simulink model "skarab_adc4x3g_14_byp"  (R2018a)
settings: Solver=VariableStepAuto  StartTime=0.0  StopTime=10.0  RelTol=1e-3
libraries: xbsIndex_r4 x140
settings Model: Creator=aisaacson  LastModifiedBy=clifford

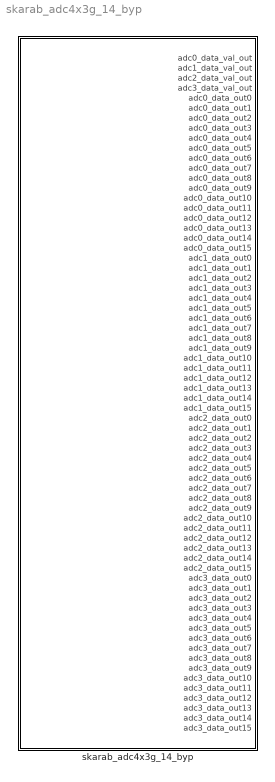
== system skarab_adc4x3g_14_byp ==
  skarab_adc4x3g_14_byp : Subsystem  Tag=xps:skarab_adc4x3g_14_byp  mask(hmc){mez=2, sync_ms=Master}
      mask prompts: mez "Mezzanine slot"; sync_ms "Master/Slave"
      mask help: Interface to ADC cards available on SKARAB boards.
      mask init:
      | skarab_adc4x3g_14_byp_mask(gcb);
      mask TypeOptions mez: 0 | 1 | 2 | 3
      mask TypeOptions sync_ms: Master | Slave
      mask DialogControl Container6 Prompt: Parameters

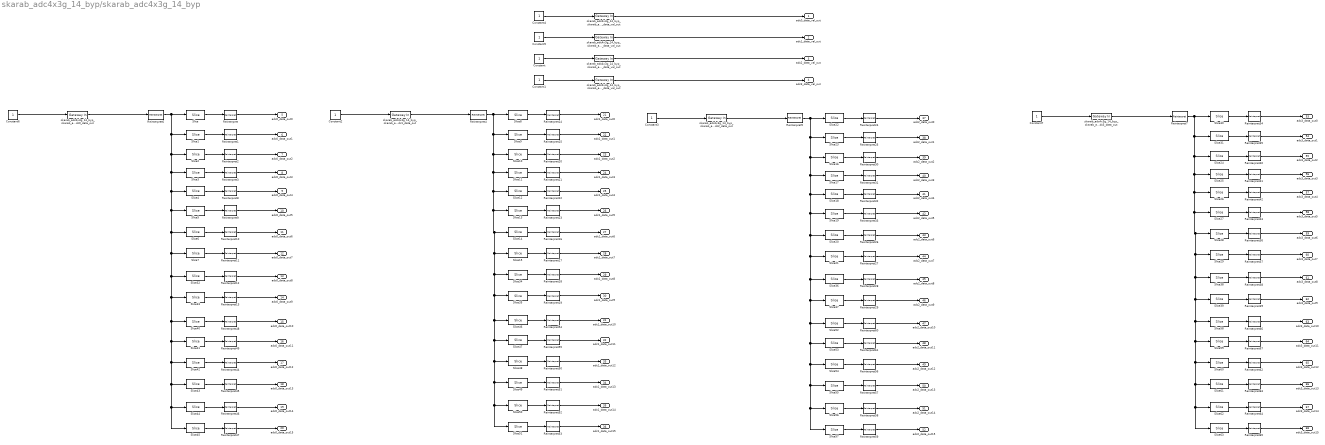
== system skarab_adc4x3g_14_byp/skarab_adc4x3g_14_byp ==
  Constant{,1..7} (8 alike) : Constant
  Reinterpret{,1..3,8..67} (64 alike) : xbsIndex_r4/Reinterpret  force_arith_type=on  arith_type="Signed  (2's comp)"  force_bin_pt=on  bin_pt=11  block_type=reinterpret
  Reinterpret{4..7} (4 alike) : xbsIndex_r4/Reinterpret  force_arith_type=on  arith_type=Unsigned  force_bin_pt=on  bin_pt=0  block_type=reinterpret
  Slice{,8,22,30} (4 alike) : xbsIndex_r4/Slice  nbits=12  boolean_output=off  mode=Lower Bit Location + Width  bit1=0  base1=MSB of Input  bit0=0  base0=LSB of Input  dbl_ovrd=off  block_type=slice
  Slice{1,9,23,31} (4 alike) : xbsIndex_r4/Slice  nbits=12  boolean_output=off  mode=Lower Bit Location + Width  bit1=0  base1=MSB of Input  bit0=12  base0=LSB of Input  dbl_ovrd=off  block_type=slice
  Slice{2,10,16,24} (4 alike) : xbsIndex_r4/Slice  nbits=12  boolean_output=off  mode=Lower Bit Location + Width  bit1=0  base1=MSB of Input  bit0=24  base0=LSB of Input  dbl_ovrd=off  block_type=slice
  Slice{3,11,17,25} (4 alike) : xbsIndex_r4/Slice  nbits=12  boolean_output=off  mode=Lower Bit Location + Width  bit1=0  base1=MSB of Input  bit0=36  base0=LSB of Input  dbl_ovrd=off  block_type=slice
  Slice{4,12,18,26} (4 alike) : xbsIndex_r4/Slice  nbits=12  boolean_output=off  mode=Lower Bit Location + Width  bit1=0  base1=MSB of Input  bit0=48  base0=LSB of Input  dbl_ovrd=off  block_type=slice
  Slice{5,13,19,27} (4 alike) : xbsIndex_r4/Slice  nbits=12  boolean_output=off  mode=Lower Bit Location + Width  bit1=0  base1=MSB of Input  bit0=60  base0=LSB of Input  dbl_ovrd=off  block_type=slice
  Slice{6,14,20,28} (4 alike) : xbsIndex_r4/Slice  nbits=12  boolean_output=off  mode=Lower Bit Location + Width  bit1=0  base1=MSB of Input  bit0=72  base0=LSB of Input  dbl_ovrd=off  block_type=slice
  Slice{7,15,21,29} (4 alike) : xbsIndex_r4/Slice  nbits=12  boolean_output=off  mode=Lower Bit Location + Width  bit1=0  base1=MSB of Input  bit0=84  base0=LSB of Input  dbl_ovrd=off  block_type=slice
  Slice{32,34,36,38} (4 alike) : xbsIndex_r4/Slice  nbits=12  boolean_output=off  mode=Lower Bit Location + Width  bit1=0  base1=MSB of Input  bit0=96  base0=LSB of Input  dbl_ovrd=off  block_type=slice
  Slice{33,35,37,39} (4 alike) : xbsIndex_r4/Slice  nbits=12  boolean_output=off  mode=Lower Bit Location + Width  bit1=0  base1=MSB of Input  bit0=108  base0=LSB of Input  dbl_ovrd=off  block_type=slice
  Slice{40,46,52,58} (4 alike) : xbsIndex_r4/Slice  nbits=12  boolean_output=off  mode=Lower Bit Location + Width  bit1=0  base1=MSB of Input  bit0=120  base0=LSB of Input  dbl_ovrd=off  block_type=slice
  Slice{41,47,53,59} (4 alike) : xbsIndex_r4/Slice  nbits=12  boolean_output=off  mode=Lower Bit Location + Width  bit1=0  base1=MSB of Input  bit0=132  base0=LSB of Input  dbl_ovrd=off  block_type=slice
  Slice{42,48,54,60} (4 alike) : xbsIndex_r4/Slice  nbits=12  boolean_output=off  mode=Lower Bit Location + Width  bit1=0  base1=MSB of Input  bit0=144  base0=LSB of Input  dbl_ovrd=off  block_type=slice
  Slice{43,49,55,61} (4 alike) : xbsIndex_r4/Slice  nbits=12  boolean_output=off  mode=Lower Bit Location + Width  bit1=0  base1=MSB of Input  bit0=156  base0=LSB of Input  dbl_ovrd=off  block_type=slice
  Slice{44,50,56,62} (4 alike) : xbsIndex_r4/Slice  nbits=12  boolean_output=off  mode=Lower Bit Location + Width  bit1=0  base1=MSB of Input  bit0=168  base0=LSB of Input  dbl_ovrd=off  block_type=slice
  Slice{45,51,57,63} (4 alike) : xbsIndex_r4/Slice  nbits=12  boolean_output=off  mode=Lower Bit Location + Width  bit1=0  base1=MSB of Input  bit0=180  base0=LSB of Input  dbl_ovrd=off  block_type=slice
  skarab_adc4x3g_14_byp_skarab_adc4x3g_14_byp_adc0_data_out : xbsIndex_r4/Gateway In  gui_display_data_type=Fixed-point  arith_type=Unsigned  n_bits=192  bin_pt=0  preci_type=Single  exp_width=8  frac_width=24  rows=1  columns=1  quantization=Truncate  overflow=Wrap  period=1  UseAsADC=off  ADCChannel='1'  interface=None  automatic_assignment=on  address_offset=hex2dec('00')  intf_name=''  intf_description=''  default_value=0  timing_constraint=None  locs_specified=off  LOCs={}  io_standard={}  inherit_from_input=off  hdl_port=on  dbl_ovrd=off  block_type=gatewayin
  skarab_adc4x3g_14_byp_skarab_adc4x3g_14_byp_adc0_data_val_out : xbsIndex_r4/Gateway In  gui_display_data_type=Boolean  arith_type=Boolean  n_bits=16  bin_pt=14  preci_type=Single  exp_width=8  frac_width=24  rows=1  columns=1  quantization="Round  (unbiased: +/- Inf)"  overflow=Saturate  period=1  UseAsADC=off  ADCChannel='1'  interface=None  automatic_assignment=on  address_offset=hex2dec('00')  intf_name=''  intf_description=''  default_value=0  timing_constraint=None  locs_specified=off  LOCs={}  io_standard={}  inherit_from_input=off  hdl_port=on  dbl_ovrd=off  block_type=gatewayin
  skarab_adc4x3g_14_byp_skarab_adc4x3g_14_byp_adc1_data_out : xbsIndex_r4/Gateway In  gui_display_data_type=Fixed-point  arith_type=Unsigned  n_bits=192  bin_pt=0  preci_type=Single  exp_width=8  frac_width=24  rows=1  columns=1  quantization=Truncate  overflow=Wrap  period=1  UseAsADC=off  ADCChannel='1'  interface=None  automatic_assignment=on  address_offset=hex2dec('00')  intf_name=''  intf_description=''  default_value=0  timing_constraint=None  locs_specified=off  LOCs={}  io_standard={}  inherit_from_input=off  hdl_port=on  dbl_ovrd=off  block_type=gatewayin
  skarab_adc4x3g_14_byp_skarab_adc4x3g_14_byp_adc1_data_val_out : xbsIndex_r4/Gateway In  gui_display_data_type=Boolean  arith_type=Boolean  n_bits=16  bin_pt=14  preci_type=Single  exp_width=8  frac_width=24  rows=1  columns=1  quantization="Round  (unbiased: +/- Inf)"  overflow=Saturate  period=1  UseAsADC=off  ADCChannel='1'  interface=None  automatic_assignment=on  address_offset=hex2dec('00')  intf_name=''  intf_description=''  default_value=0  timing_constraint=None  locs_specified=off  LOCs={}  io_standard={}  inherit_from_input=off  hdl_port=on  dbl_ovrd=off  block_type=gatewayin
  skarab_adc4x3g_14_byp_skarab_adc4x3g_14_byp_adc2_data_out : xbsIndex_r4/Gateway In  gui_display_data_type=Fixed-point  arith_type=Unsigned  n_bits=192  bin_pt=0  preci_type=Single  exp_width=8  frac_width=24  rows=1  columns=1  quantization=Truncate  overflow=Wrap  period=1  UseAsADC=off  ADCChannel='1'  interface=None  automatic_assignment=on  address_offset=hex2dec('00')  intf_name=''  intf_description=''  default_value=0  timing_constraint=None  locs_specified=off  LOCs={}  io_standard={}  inherit_from_input=off  hdl_port=on  dbl_ovrd=off  block_type=gatewayin
  skarab_adc4x3g_14_byp_skarab_adc4x3g_14_byp_adc2_data_val_out : xbsIndex_r4/Gateway In  gui_display_data_type=Boolean  arith_type=Boolean  n_bits=16  bin_pt=14  preci_type=Single  exp_width=8  frac_width=24  rows=1  columns=1  quantization="Round  (unbiased: +/- Inf)"  overflow=Saturate  period=1  UseAsADC=off  ADCChannel='1'  interface=None  automatic_assignment=on  address_offset=hex2dec('00')  intf_name=''  intf_description=''  default_value=0  timing_constraint=None  locs_specified=off  LOCs={}  io_standard={}  inherit_from_input=off  hdl_port=on  dbl_ovrd=off  block_type=gatewayin
  skarab_adc4x3g_14_byp_skarab_adc4x3g_14_byp_adc3_data_out : xbsIndex_r4/Gateway In  gui_display_data_type=Fixed-point  arith_type=Unsigned  n_bits=192  bin_pt=0  preci_type=Single  exp_width=8  frac_width=24  rows=1  columns=1  quantization=Truncate  overflow=Wrap  period=1  UseAsADC=off  ADCChannel='1'  interface=None  automatic_assignment=on  address_offset=hex2dec('00')  intf_name=''  intf_description=''  default_value=0  timing_constraint=None  locs_specified=off  LOCs={}  io_standard={}  inherit_from_input=off  hdl_port=on  dbl_ovrd=off  block_type=gatewayin
  skarab_adc4x3g_14_byp_skarab_adc4x3g_14_byp_adc3_data_val_out : xbsIndex_r4/Gateway In  gui_display_data_type=Boolean  arith_type=Boolean  n_bits=16  bin_pt=14  preci_type=Single  exp_width=8  frac_width=24  rows=1  columns=1  quantization="Round  (unbiased: +/- Inf)"  overflow=Saturate  period=1  UseAsADC=off  ADCChannel='1'  interface=None  automatic_assignment=on  address_offset=hex2dec('00')  intf_name=''  intf_description=''  default_value=0  timing_constraint=None  locs_specified=off  LOCs={}  io_standard={}  inherit_from_input=off  hdl_port=on  dbl_ovrd=off  block_type=gatewayin
  adc0_data_val_out : Outport
  adc1_data_val_out : Outport  Port=2
  adc2_data_val_out : Outport  Port=3
  adc3_data_val_out : Outport  Port=4
  adc0_data_out0 : Outport  Port=5
  adc0_data_out1 : Outport  Port=6
  adc0_data_out2 : Outport  Port=7
  adc0_data_out3 : Outport  Port=8
  adc0_data_out4 : Outport  Port=9
  adc0_data_out5 : Outport  Port=10
  adc0_data_out6 : Outport  Port=11
  adc0_data_out7 : Outport  Port=12
  adc0_data_out8 : Outport  Port=13
  adc0_data_out9 : Outport  Port=14
  adc0_data_out10 : Outport  Port=15
  adc0_data_out11 : Outport  Port=16
  adc0_data_out12 : Outport  Port=17
  adc0_data_out13 : Outport  Port=18
  adc0_data_out14 : Outport  Port=19
  adc0_data_out15 : Outport  Port=20
  adc1_data_out0 : Outport  Port=21
  adc1_data_out1 : Outport  Port=22
  adc1_data_out2 : Outport  Port=23
  adc1_data_out3 : Outport  Port=24
  adc1_data_out4 : Outport  Port=25
  adc1_data_out5 : Outport  Port=26
  adc1_data_out6 : Outport  Port=27
  adc1_data_out7 : Outport  Port=28
  adc1_data_out8 : Outport  Port=29
  adc1_data_out9 : Outport  Port=30
  adc1_data_out10 : Outport  Port=31
  adc1_data_out11 : Outport  Port=32
  adc1_data_out12 : Outport  Port=33
  adc1_data_out13 : Outport  Port=34
  adc1_data_out14 : Outport  Port=35
  adc1_data_out15 : Outport  Port=36
  adc2_data_out0 : Outport  Port=37
  adc2_data_out1 : Outport  Port=38
  adc2_data_out2 : Outport  Port=39
  adc2_data_out3 : Outport  Port=40
  adc2_data_out4 : Outport  Port=41
  adc2_data_out5 : Outport  Port=42
  adc2_data_out6 : Outport  Port=43
  adc2_data_out7 : Outport  Port=44
  adc2_data_out8 : Outport  Port=45
  adc2_data_out9 : Outport  Port=46
  adc2_data_out10 : Outport  Port=47
  adc2_data_out11 : Outport  Port=48
  adc2_data_out12 : Outport  Port=49
  adc2_data_out13 : Outport  Port=50
  adc2_data_out14 : Outport  Port=51
  adc2_data_out15 : Outport  Port=52
  adc3_data_out0 : Outport  Port=53
  adc3_data_out1 : Outport  Port=54
  adc3_data_out2 : Outport  Port=55
  adc3_data_out3 : Outport  Port=56
  adc3_data_out4 : Outport  Port=57
  adc3_data_out5 : Outport  Port=58
  adc3_data_out6 : Outport  Port=59
  adc3_data_out7 : Outport  Port=60
  adc3_data_out8 : Outport  Port=61
  adc3_data_out9 : Outport  Port=62
  adc3_data_out10 : Outport  Port=63
  adc3_data_out11 : Outport  Port=64
  adc3_data_out12 : Outport  Port=65
  adc3_data_out13 : Outport  Port=66
  adc3_data_out14 : Outport  Port=67
  adc3_data_out15 : Outport  Port=68
  wires:
  Reinterpret7/1 -> Slice30/1, Slice31/1, Slice24/1, Slice25/1, Slice26/1, Slice27/1, Slice28/1, Slice29/1, Slice38/1, Slice63/1, Slice62/1, Slice61/1, Slice60/1, Slice59/1, Slice58/1, Slice39/1
  Reinterpret54/1 -> adc1_data_out10/1
  Slice7/1 -> Reinterpret11/1
  Slice55/1 -> Reinterpret57/1
  Reinterpret39/1 -> adc3_data_out9/1
  Slice62/1 -> Reinterpret64/1
  Slice28/1 -> Reinterpret36/1
  Slice22/1 -> Reinterpret24/1
  Reinterpret57/1 -> adc2_data_out13/1
  Reinterpret62/1 -> adc3_data_out12/1
  Reinterpret46/1 -> adc0_data_out14/1
  Reinterpret23/1 -> adc1_data_out5/1
  Slice57/1 -> Reinterpret59/1
  skarab_adc4x3g_14_byp_skarab_adc4x3g_14_byp_adc3_data_val_out/1 -> adc3_data_val_out/1
  Slice54/1 -> Reinterpret56/1
  Constant1/1 -> skarab_adc4x3g_14_byp_skarab_adc4x3g_14_byp_adc3_data_val_out/1
  Slice6/1 -> Reinterpret10/1
  skarab_adc4x3g_14_byp_skarab_adc4x3g_14_byp_adc1_data_out/1 -> Reinterpret4/1
  Slice50/1 -> Reinterpret52/1
  Constant/1 -> skarab_adc4x3g_14_byp_skarab_adc4x3g_14_byp_adc2_data_val_out/1
  Reinterpret30/1 -> adc2_data_out2/1
  Reinterpret47/1 -> adc0_data_out15/1
  Slice21/1 -> Reinterpret27/1
  Slice37/1 -> Reinterpret29/1
  Reinterpret49/1 -> adc0_data_out11/1
  Reinterpret14/1 -> adc1_data_out0/1
  Slice15/1 -> Reinterpret17/1
  Reinterpret10/1 -> adc0_data_out6/1
  skarab_adc4x3g_14_byp_skarab_adc4x3g_14_byp_adc2_data_val_out/1 -> adc2_data_val_out/1
  Reinterpret51/1 -> adc1_data_out13/1
  Reinterpret21/1 -> adc1_data_out3/1
  Reinterpret66/1 -> adc3_data_out10/1
  Slice34/1 -> Reinterpret18/1
  Reinterpret60/1 -> adc2_data_out10/1
  Reinterpret48/1 -> adc0_data_out10/1
  Slice59/1 -> Reinterpret67/1
  Reinterpret12/1 -> adc0_data_out8/1
  Constant4/1 -> skarab_adc4x3g_14_byp_skarab_adc4x3g_14_byp_adc0_data_val_out/1
  skarab_adc4x3g_14_byp_skarab_adc4x3g_14_byp_adc0_data_val_out/1 -> adc0_data_val_out/1
  Slice58/1 -> Reinterpret66/1
  skarab_adc4x3g_14_byp_skarab_adc4x3g_14_byp_adc0_data_out/1 -> Reinterpret6/1
  skarab_adc4x3g_14_byp_skarab_adc4x3g_14_byp_adc1_data_val_out/1 -> adc1_data_val_out/1
  Reinterpret34/1 -> adc3_data_out0/1
  Slice11/1 -> Reinterpret21/1
  Slice5/1 -> Reinterpret9/1
  Slice35/1 -> Reinterpret19/1
  Slice4/1 -> Reinterpret8/1
  Reinterpret9/1 -> adc0_data_out5/1
  Reinterpret/1 -> adc0_data_out0/1
  Constant2/1 -> skarab_adc4x3g_14_byp_skarab_adc4x3g_14_byp_adc1_data_out/1
  Reinterpret11/1 -> adc0_data_out7/1
  Slice23/1 -> Reinterpret25/1
  Slice10/1 -> Reinterpret20/1
  Slice45/1 -> Reinterpret47/1
  Slice42/1 -> Reinterpret44/1
  Reinterpret36/1 -> adc3_data_out6/1
  Slice60/1 -> Reinterpret62/1
  Reinterpret19/1 -> adc1_data_out9/1
  Slice14/1 -> Reinterpret16/1
  Constant6/1 -> skarab_adc4x3g_14_byp_skarab_adc4x3g_14_byp_adc0_data_out/1
  Reinterpret35/1 -> adc3_data_out1/1
  skarab_adc4x3g_14_byp_skarab_adc4x3g_14_byp_adc2_data_out/1 -> Reinterpret5/1
  Slice43/1 -> Reinterpret45/1
  Slice30/1 -> Reinterpret34/1
  Slice41/1 -> Reinterpret49/1
  Reinterpret1/1 -> adc0_data_out1/1
  Reinterpret56/1 -> adc2_data_out12/1
  Slice46/1 -> Reinterpret54/1
  Reinterpret58/1 -> adc2_data_out14/1
  Reinterpret16/1 -> adc1_data_out6/1
  Slice24/1 -> Reinterpret40/1
  Reinterpret37/1 -> adc3_data_out7/1
  Constant3/1 -> skarab_adc4x3g_14_byp_skarab_adc4x3g_14_byp_adc2_data_out/1
  Reinterpret5/1 -> Slice22/1, Slice23/1, Slice16/1, Slice17/1, Slice18/1, Slice19/1, Slice20/1, Slice21/1, Slice36/1, Slice57/1, Slice56/1, Slice55/1, Slice54/1, Slice53/1, Slice52/1, Slice37/1
  Slice12/1 -> Reinterpret22/1
  Slice32/1 -> Reinterpret12/1
  Slice13/1 -> Reinterpret23/1
  Reinterpret41/1 -> adc3_data_out3/1
  Reinterpret15/1 -> adc1_data_out1/1
  Reinterpret17/1 -> adc1_data_out7/1
  Reinterpret40/1 -> adc3_data_out2/1
  Slice33/1 -> Reinterpret13/1
  Reinterpret45/1 -> adc0_data_out13/1
  Reinterpret28/1 -> adc2_data_out8/1
  Reinterpret42/1 -> adc3_data_out4/1
  Slice38/1 -> Reinterpret38/1
  Reinterpret38/1 -> adc3_data_out8/1
  Reinterpret22/1 -> adc1_data_out4/1
  Reinterpret43/1 -> adc3_data_out5/1
  Reinterpret25/1 -> adc2_data_out1/1
  Slice2/1 -> Reinterpret2/1
  Reinterpret63/1 -> adc3_data_out13/1
  Slice31/1 -> Reinterpret35/1
  Reinterpret6/1 -> Slice/1, Slice1/1, Slice2/1, Slice3/1, Slice4/1, Slice5/1, Slice6/1, Slice7/1, Slice32/1, Slice45/1, Slice44/1, Slice43/1, Slice42/1, Slice41/1, Slice40/1, Slice33/1
  Slice27/1 -> Reinterpret43/1
  Slice52/1 -> Reinterpret60/1
  Slice39/1 -> Reinterpret39/1
  Slice29/1 -> Reinterpret37/1
  Reinterpret20/1 -> adc1_data_out2/1
  Constant5/1 -> skarab_adc4x3g_14_byp_skarab_adc4x3g_14_byp_adc1_data_val_out/1
  Slice16/1 -> Reinterpret30/1
  Slice8/1 -> Reinterpret14/1
  Slice9/1 -> Reinterpret15/1
  Reinterpret53/1 -> adc1_data_out15/1
  Reinterpret29/1 -> adc2_data_out9/1
  Slice25/1 -> Reinterpret41/1
  Slice/1 -> Reinterpret/1
  Slice51/1 -> Reinterpret53/1
  Slice44/1 -> Reinterpret46/1
  Reinterpret3/1 -> adc0_data_out3/1
  Reinterpret67/1 -> adc3_data_out11/1
  Slice47/1 -> Reinterpret55/1
  Reinterpret2/1 -> adc0_data_out2/1
  skarab_adc4x3g_14_byp_skarab_adc4x3g_14_byp_adc3_data_out/1 -> Reinterpret7/1
  Reinterpret18/1 -> adc1_data_out8/1
  Reinterpret27/1 -> adc2_data_out7/1
  Slice20/1 -> Reinterpret26/1
  Slice1/1 -> Reinterpret1/1
  Slice63/1 -> Reinterpret65/1
  Reinterpret26/1 -> adc2_data_out6/1
  Slice18/1 -> Reinterpret32/1
  Reinterpret13/1 -> adc0_data_out9/1
  Slice19/1 -> Reinterpret33/1
  Slice48/1 -> Reinterpret50/1
  Slice26/1 -> Reinterpret42/1
  Reinterpret33/1 -> adc2_data_out5/1
  Slice56/1 -> Reinterpret58/1
  Reinterpret65/1 -> adc3_data_out15/1
  Reinterpret4/1 -> Slice8/1, Slice9/1, Slice10/1, Slice11/1, Slice12/1, Slice13/1, Slice14/1, Slice15/1, Slice51/1, Slice50/1, Slice49/1, Slice48/1, Slice47/1, Slice46/1, Slice35/1, Slice34/1
  Reinterpret44/1 -> adc0_data_out12/1
  Slice40/1 -> Reinterpret48/1
  Slice61/1 -> Reinterpret63/1
  Reinterpret50/1 -> adc1_data_out12/1
  Slice49/1 -> Reinterpret51/1
  Slice17/1 -> Reinterpret31/1
  Reinterpret64/1 -> adc3_data_out14/1
  Slice36/1 -> Reinterpret28/1
  Reinterpret55/1 -> adc1_data_out11/1
  Reinterpret59/1 -> adc2_data_out15/1
  Slice3/1 -> Reinterpret3/1
  Constant7/1 -> skarab_adc4x3g_14_byp_skarab_adc4x3g_14_byp_adc3_data_out/1
  Reinterpret31/1 -> adc2_data_out3/1
  Reinterpret24/1 -> adc2_data_out0/1
  Reinterpret61/1 -> adc2_data_out11/1
  Slice53/1 -> Reinterpret61/1
  Reinterpret52/1 -> adc1_data_out14/1
  Reinterpret32/1 -> adc2_data_out4/1
  Reinterpret8/1 -> adc0_data_out4/1
